simulink model "half_wave_RL_freewheel"  (R2024b)
settings: Solver=ode23tb  StartTime=0.0  StopTime=0.1  MaxStep=1e-5  RelTol=1e-3
model workspace (MAT data in the model file):
  L_load = 0.5
  R_load = 50
  U2_rms = 220
  alpha_deg = 30
  freq_hz = 50
libraries: spsVoltageMeasurementLib x3, spsACVoltageSourceLib x1, spsCurrentMeasurementLib x1, spsDiodeLib x1, spsSeriesRLCBranchLib x1, spsThyristorLib x1, spspowerguiLib x1
settings Model: Creator=l2001  LastModifiedBy=l2001

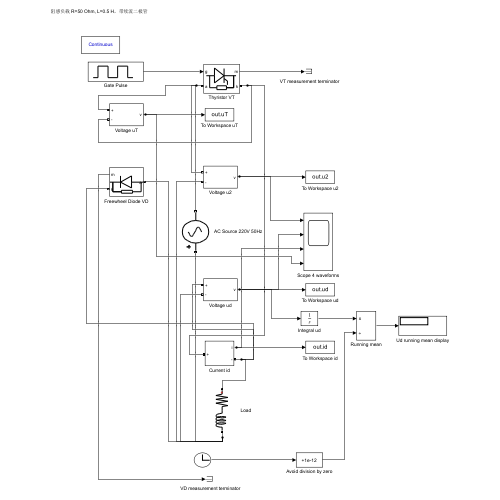
[thumbnail: Simulink's stored preview of the top-level diagram]
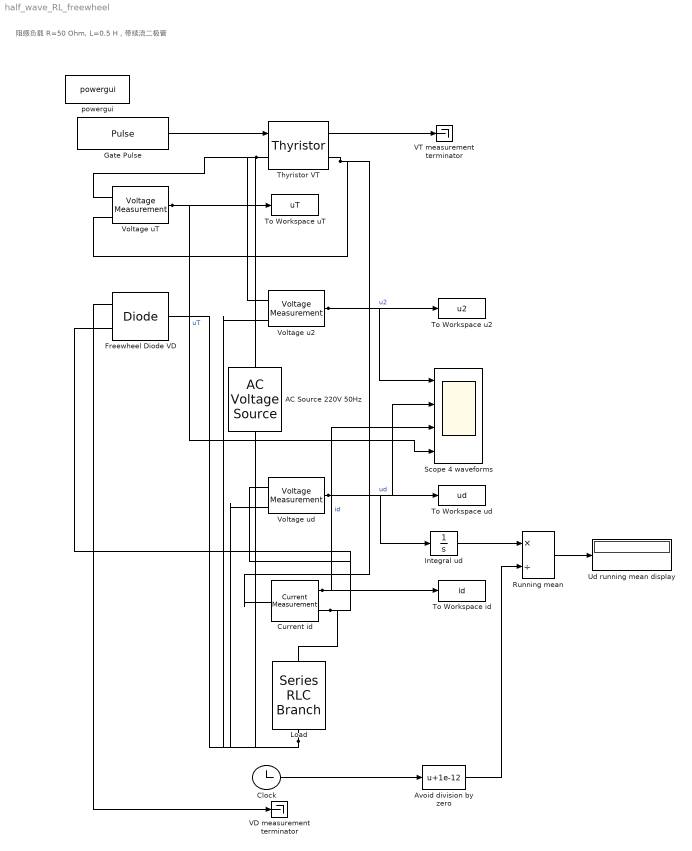
== system half_wave_RL_freewheel ==
  note: 阻感负载 R=50 Ohm, L=0.5 H，带续流二极管
  AC Source 220V 50Hz : spsACVoltageSourceLib/AC Voltage Source  Amplitude=sqrt(2)*U2_rms  Phase=0  Frequency=freq_hz  SampleTime=0  Measurements=None  BusType=swing  Pref=10e3  Qref=0  Qmin=-inf  Qmax=+inf
  Avoid division by zero : Bias  Bias=1e-12  SaturateOnIntegerOverflow=off
  Clock : Clock
  Current id : spsCurrentMeasurementLib/Current Measurement  PhasorSimulation=off  OutputType=Complex  PSBequivalent=0
  Freewheel Diode VD : spsDiodeLib/Diode  Ron=0.001  Lon=0  Vf=0.8  IC=0  UseSnubber=0  Rs=500  Cs=250e-9  Measurements=on
  Gate Pulse : DiscretePulseGenerator  PulseType=Time based  Period=1/freq_hz  PulseWidth=5  PhaseDelay=alpha_deg/360/freq_hz  SampleTime=0
  Integral ud : Integrator
  Load : spsSeriesRLCBranchLib/Series RLC Branch  LConnTagsString=__new0  RConnTagsString=__new0  BranchType=RL  Resistance=R_load  Inductance=L_load  SetiL0=on  InitialCurrent=0  Capacitance=1e-6  Setx0=off  InitialVoltage=0  Measurements=None
  Running mean : Product  Inputs=*/
  Scope 4 waveforms : Scope  NumInputPorts=4
  Thyristor VT : spsThyristorLib/Thyristor  Ron=0.001  Lon=0  Vf=0.8  IC=0  Rs=500  Cs=250e-9  Measurements=on
  To Workspace id : ToWorkspace  VariableName=id  SaveFormat=Timeseries  SampleTime=-1
  To Workspace u2 : ToWorkspace  VariableName=u2  SaveFormat=Timeseries  SampleTime=-1
  To Workspace uT : ToWorkspace  VariableName=uT  SaveFormat=Timeseries  SampleTime=-1
  To Workspace ud : ToWorkspace  VariableName=ud  SaveFormat=Timeseries  SampleTime=-1
  Ud running mean display : Display
  VD measurement terminator : Terminator
  VT measurement terminator : Terminator
  Voltage u2 : spsVoltageMeasurementLib/Voltage Measurement  PhasorSimulation=off  OutputType=Complex  PSBequivalent=0
  Voltage uT : spsVoltageMeasurementLib/Voltage Measurement  PhasorSimulation=off  OutputType=Complex  PSBequivalent=0
  Voltage ud : spsVoltageMeasurementLib/Voltage Measurement  PhasorSimulation=off  OutputType=Complex  PSBequivalent=0
  powergui : spspowerguiLib/powergui  Priority=1  SimulationMode=Continuous  SampleTime=50e-6  frequency=60  Iterations=50  frequencyindice=60  Pbase=100e6  ErrMax=1e-4  UnitsV=kV  UnitsW=MW  buscounter=0  FunctionMessages=off  echomessages=off  EnableUseOfTLC=off  CurrentSourceSwitches=off  DisableSnubberDevices=off  DisableRonSwitches=off  DisableVfSwitches=off  DisplayEquations=off  AutomaticDiscreteSolvers=off  SolverType=Tustin/Backward Euler (TBE)  Interpol=off  ExternalGateDelay=off  methode=off  Ts=100  x0status=blocks  SPID=on  SwTol=0  HookPort=off  NonlinearTolerance=1e-4  nMaxIteration=100  ContinueOnMaxIteration=off  RestoreLinks=warning  ResistiveCurrentMeasurement=off  Frange=[0:2:500]  Ylog=off  Xlog=on  ShowGrid=off  save=off  variable=ZData  structure=0  ZoomFFT=off  StartTime=0.0  cycles=1  DisplayStyle=1  fundamental=60  FreqAxis=off  MaxFrequency=1000  frequencyindicesteady=1  RmsSteady=1  display=off
  wires:
  Freewheel Diode VD/1 -> VD measurement terminator/1
  Gate Pulse/1 -> Thyristor VT/1
  Avoid division by zero/1 -> Running mean/2
  Voltage uT/1 -> Scope 4 waveforms/4, To Workspace uT/1  "uT"
  Thyristor VT/1 -> VT measurement terminator/1
  Voltage u2/1 -> Scope 4 waveforms/1, To Workspace u2/1  "u2"
  Voltage ud/1 -> To Workspace ud/1, Scope 4 waveforms/2, Integral ud/1  "ud"
  Current id/1 -> To Workspace id/1, Scope 4 waveforms/3  "id"
  Clock/1 -> Avoid division by zero/1
  Integral ud/1 -> Running mean/1
  Running mean/1 -> Ud running mean display/1
  connections:
  Voltage uT/LConn2 -- Current id/LConn1 -- Thyristor VT/RConn1
  Voltage uT/LConn1 -- AC Source 220V 50Hz/LConn1 -- Voltage u2/LConn1 -- Thyristor VT/LConn1
  Freewheel Diode VD/LConn1 -- AC Source 220V 50Hz/RConn1 -- Voltage ud/LConn2 -- Voltage u2/LConn2 -- Load/RConn1
  Freewheel Diode VD/RConn1 -- Voltage ud/LConn1 -- Current id/RConn1 -- Load/LConn1
